simulink model "power_limiter_A_test"  (R2018b)
settings: Solver=VariableStepAuto  StartTime=0.0  StopTime=110  RelTol=1e-3
PreLoadFcn:
  | load_system('../simulink_reference_models/test_sequence_lib');
InitFcn:
  | close all
  | clear all
  | 
  | T_CNTL = 1/5e3;
  | 
  | P_NOM = 1e6;
  | VLL_NOM = 480;
  | I_BASE = P_NOM / (sqrt(3) * VLL_NOM);
  | F_NOM = 60;
  | W_NOM = 2 * 3.14159265 * F_NOM;
  | 
  | Z_BASE = VLL_NOM * VLL_NOM / P_NOM;
  | L_BASE = Z_BASE / W_NOM;
  | C_BASE = 1 / (W_NOM * Z_BASE);
libraries: simulink x16, test_sequence_lib x4
settings Model: SimulationMode=rapid-accelerator  Creator=HussamAlatrash  LastModifiedBy=ahhei
settings DataIOCC: ReturnWorkspaceOutputs=on
settings DebuggingCC: UnconnectedInputMsg=none  UnconnectedOutputMsg=none  UnconnectedLineMsg=none
settings ModelReferenceCC: EnableRefExpFcnMdlSchedulingChecks=off
settings RTWCC: Description=Generic Real-Time Target
settings ConfigComp: CovBoundaryAbsTol=1.0e-5

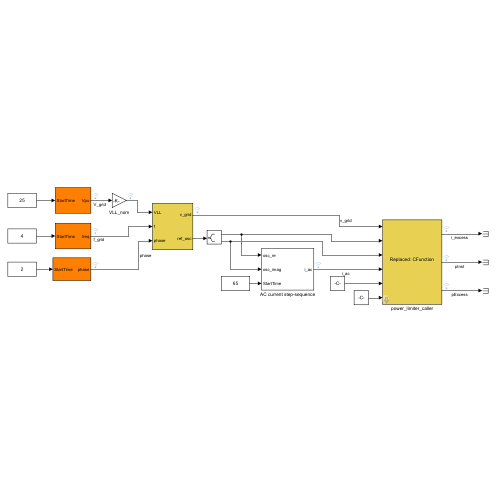
[thumbnail: Simulink's stored preview of the top-level diagram]
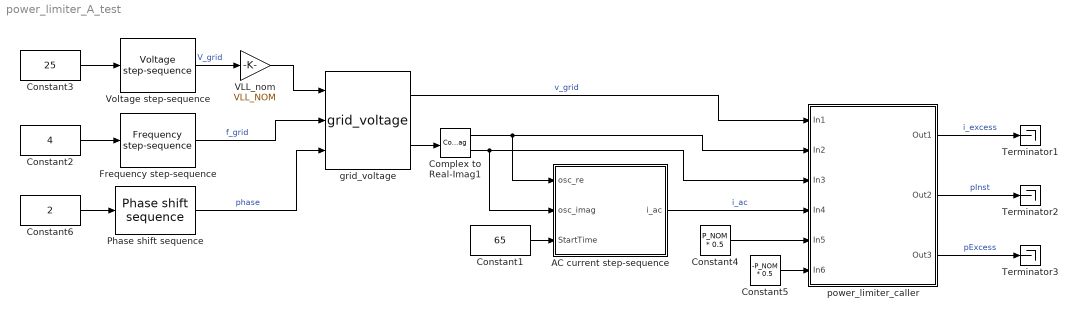
== system power_limiter_A_test ==
  AC current step-sequence : Subsystem
  Complex to Real-Imag1 : ComplexToRealImag
  Constant1 : Constant  Value=65
  Constant2 : Constant  Value=4
  Constant3 : Constant  Value=25
  Constant4 : Constant  Value=P_NOM * 0.5
  Constant5 : Constant  Value=-P_NOM * 0.5
  Constant6 : Constant  Value=2
  Frequency step-sequence : test_sequence_lib/Frequency step-sequence  SystemSampleTime=-1  EmptyChoice=off  PassThrough=off  PassThroughVariantControl=(default)  EmptyChoiceVariantControl=(default)  Latency=0  AutoFrameSizeCalculation=off
  Phase shift sequence : test_sequence_lib/Phase shift sequence  SystemSampleTime=-1  EmptyChoice=off  PassThrough=off  PassThroughVariantControl=(default)  EmptyChoiceVariantControl=(default)  Latency=0  AutoFrameSizeCalculation=off
  Terminator1 : Terminator
  Terminator2 : Terminator
  Terminator3 : Terminator
  VLL_nom : Gain  Gain=VLL_NOM
  Voltage step-sequence : test_sequence_lib/Voltage step-sequence  SystemSampleTime=-1  EmptyChoice=off  PassThrough=off  PassThroughVariantControl=(default)  EmptyChoiceVariantControl=(default)  Latency=0  AutoFrameSizeCalculation=off
  grid_voltage : test_sequence_lib/grid_voltage  SystemSampleTime=-1  EmptyChoice=off  PassThrough=off  PassThroughVariantControl=(default)  EmptyChoiceVariantControl=(default)  Latency=0  AutoFrameSizeCalculation=off
  power_limiter_caller : Subsystem  Description=Replaced Block  mask(Replaced Block){}
      mask help: This block has been replaced with an empty subsystem because it used functionality that is unavailable in Simulink R2018b.
      mask Display: fprintf('Replaced: %s\n','CFunction')
  wires:
  Constant2/1 -> Frequency step-sequence/1
  Constant3/1 -> Voltage step-sequence/1
  grid_voltage/1 -> power_limiter_caller/1(In1)  "v_grid"
  Constant6/1 -> Phase shift sequence/1
  VLL_nom/1 -> grid_voltage/1
  grid_voltage/2 -> Complex to Real-Imag1/1
  power_limiter_caller/1(Out1) -> Terminator1/1  "i_excess"
  power_limiter_caller/2(Out2) -> Terminator2/1  "pInst"
  power_limiter_caller/3(Out3) -> Terminator3/1  "pExcess"
  Voltage step-sequence/1 -> VLL_nom/1  "V_grid"
  Frequency step-sequence/1 -> grid_voltage/2  "f_grid"
  Phase shift sequence/1 -> grid_voltage/3  "phase"
  Constant5/1 -> power_limiter_caller/6(In6)
  Constant4/1 -> power_limiter_caller/5(In5)
  Constant1/1 -> AC current step-sequence/3(StartTime)
  Complex to Real-Imag1/1 -> AC current step-sequence/1(osc_re), power_limiter_caller/2(In2)
  Complex to Real-Imag1/2 -> AC current step-sequence/2(osc_imag), power_limiter_caller/3(In3)
  AC current step-sequence/1(i_ac) -> power_limiter_caller/4(In4)  "i_ac"

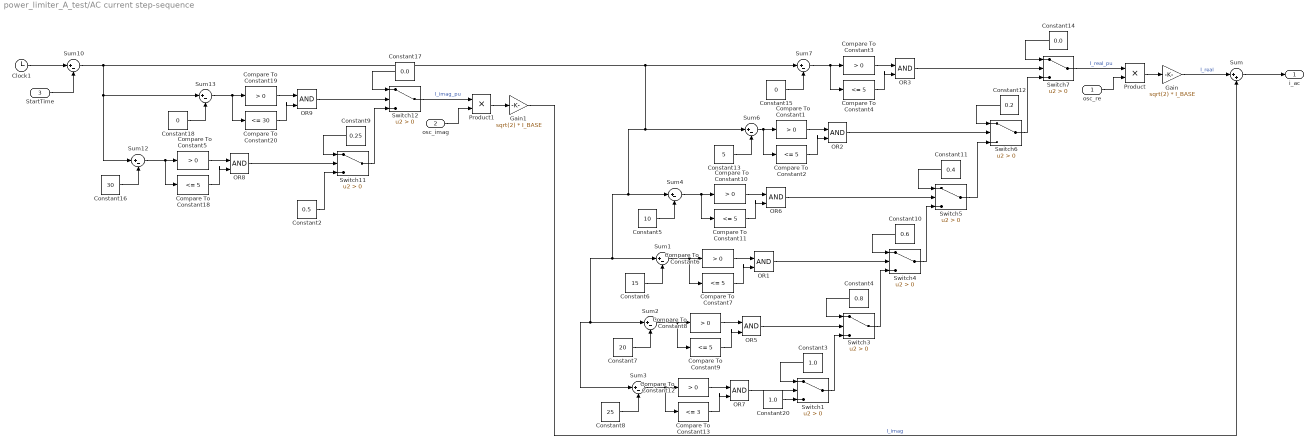
== system power_limiter_A_test/AC current step-sequence ==
  osc_re : Inport
  osc_imag : Inport  Port=2
  StartTime : Inport  Port=3
  Clock1 : Clock
  Compare To Constant{1,3,5..6,8,10,12,19} (8 alike) : simulink/Logic and Bit Operations/Compare To Constant  relop=>  const=0  OutDataTypeStr=boolean
  Compare To Constant{2,4,7,9,11,18} (6 alike) : simulink/Logic and Bit Operations/Compare To Constant  relop=<=  const=5  OutDataTypeStr=boolean
  Compare To Constant13 : simulink/Logic and Bit Operations/Compare To Constant  relop=<=  const=3  OutDataTypeStr=boolean
  Compare To Constant20 : simulink/Logic and Bit Operations/Compare To Constant  relop=<=  const=30  OutDataTypeStr=boolean
  Constant10 : Constant  Value=0.6
  Constant11 : Constant  Value=0.4
  Constant12 : Constant  Value=0.2
  Constant13 : Constant  Value=5
  Constant14 : Constant  Value=0.0
  Constant15 : Constant  Value=0
  Constant16 : Constant  Value=30
  Constant17 : Constant  Value=0.0
  Constant18 : Constant  Value=0
  Constant2 : Constant  Value=0.5
  Constant20 : Constant  Value=1.0
  Constant3 : Constant  Value=1.0
  Constant4 : Constant  Value=0.8
  Constant5 : Constant  Value=10
  Constant6 : Constant  Value=15
  Constant7 : Constant  Value=20
  Constant8 : Constant  Value=25
  Constant9 : Constant  Value=0.25
  Gain : Gain  Gain=sqrt(2) * I_BASE
  Gain1 : Gain  Gain=sqrt(2) * I_BASE
  OR{1..3,5..9} (8 alike) : Logic  IconShape=distinctive  AllPortsSameDT=off  OutDataTypeStr=boolean
  Product : Product
  Product1 : Product
  Sum : Sum  Inputs=|++
  Sum{1..4,6..7,10,12..13} (9 alike) : Sum  Inputs=|+-
  Switch{1,3..7,11..12} (8 alike) : Switch  Criteria=u2 > Threshold
  i_ac : Outport
  wires:
  StartTime/1 -> Sum10/2
  Clock1/1 -> Sum10/1
  Switch7/1 -> Product/1  "I_real_pu"
  Switch6/1 -> Switch7/3
  Constant14/1 -> Switch7/1
  Compare To Constant4/1 -> OR3/2
  Compare To Constant3/1 -> OR3/1
  OR3/1 -> Switch7/2
  Constant15/1 -> Sum7/2
  Sum7/1 -> Compare To Constant4/1, Compare To Constant3/1
  Sum6/1 -> Compare To Constant1/1, Compare To Constant2/1
  Constant13/1 -> Sum6/2
  OR2/1 -> Switch6/2
  Compare To Constant1/1 -> OR2/1
  Compare To Constant2/1 -> OR2/2
  Constant12/1 -> Switch6/1
  Switch5/1 -> Switch6/3
  Switch4/1 -> Switch5/3
  Switch3/1 -> Switch4/3
  Switch1/1 -> Switch3/3
  Constant11/1 -> Switch5/1
  Constant10/1 -> Switch4/1
  OR1/1 -> Switch4/2
  OR5/1 -> Switch3/2
  Constant4/1 -> Switch3/1
  Sum3/1 -> Compare To Constant12/1, Compare To Constant13/1
  Constant8/1 -> Sum3/2
  Compare To Constant12/1 -> OR7/1
  Compare To Constant13/1 -> OR7/2
  Compare To Constant9/1 -> OR5/2
  Compare To Constant8/1 -> OR5/1
  Constant7/1 -> Sum2/2
  Sum2/1 -> Compare To Constant9/1, Compare To Constant8/1
  Sum1/1 -> Compare To Constant6/1, Compare To Constant7/1
  Constant6/1 -> Sum1/2
  Compare To Constant6/1 -> OR1/1
  Compare To Constant7/1 -> OR1/2
  Compare To Constant11/1 -> OR6/2
  Compare To Constant10/1 -> OR6/1
  OR6/1 -> Switch5/2
  Constant5/1 -> Sum4/2
  Sum4/1 -> Compare To Constant11/1, Compare To Constant10/1
  Constant3/1 -> Switch1/1
  OR7/1 -> Switch1/2
  Constant20/1 -> Switch1/3
  osc_re/1 -> Product/2
  Product/1 -> Gain/1
  Constant9/1 -> Switch11/1
  Switch11/1 -> Switch12/3
  Sum10/1 -> Sum12/1, Sum13/1, Sum7/1, Sum2/1, Sum3/1, Sum1/1, Sum4/1, Sum6/1
  Sum12/1 -> Compare To Constant5/1, Compare To Constant18/1
  Constant17/1 -> Switch12/1
  Compare To Constant19/1 -> OR9/1
  OR8/1 -> Switch11/2
  Compare To Constant20/1 -> OR9/2
  Compare To Constant18/1 -> OR8/2
  Compare To Constant5/1 -> OR8/1
  Constant2/1 -> Switch11/3
  Constant16/1 -> Sum12/2
  Sum13/1 -> Compare To Constant20/1, Compare To Constant19/1
  Switch12/1 -> Product1/1  "I_imag_pu"
  Constant18/1 -> Sum13/2
  OR9/1 -> Switch12/2
  Product1/1 -> Gain1/1
  osc_imag/1 -> Product1/2
  Gain/1 -> Sum/1  "I_real"
  Gain1/1 -> Sum/2  "I_imag"
  Sum/1 -> i_ac/1

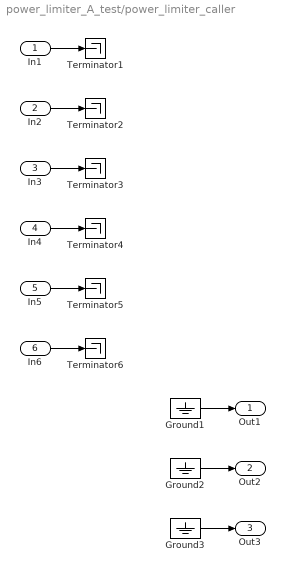
== system power_limiter_A_test/power_limiter_caller ==
  In1 : Inport
  In2 : Inport  Port=2
  In3 : Inport  Port=3
  In4 : Inport  Port=4
  In5 : Inport  Port=5
  In6 : Inport  Port=6
  Ground1 : Ground
  Ground2 : Ground
  Ground3 : Ground
  Terminator{1..6} (6 alike) : Terminator
  Out1 : Outport
  Out2 : Outport  Port=2
  Out3 : Outport  Port=3
  wires:
  Ground3/1 -> Out3/1
  Ground2/1 -> Out2/1
  Ground1/1 -> Out1/1
  In6/1 -> Terminator6/1
  In5/1 -> Terminator5/1
  In4/1 -> Terminator4/1
  In3/1 -> Terminator3/1
  In2/1 -> Terminator2/1
  In1/1 -> Terminator1/1
